simulink model "EvitarObstaculo"  (R2023b)
settings: Solver=FixedStepAuto  StartTime=0.0  StopTime=100.0  FixedStep=Ts  RelTol=1e-3
values from neighbouring files (symbols this model uses):
  obsx = 2    [EjecutarEsquivarObs.m]    (also in EjecutarEsquivarObs_traj.m = 1.75)
  obsy = 0    [EjecutarEsquivarObs.m]    (also in EjecutarEsquivarObs_traj.m = 0.7)
  refx = 10*rand-5    [EjecutarBorroso.m]    (also in EjecutarEsquivarObs.m = 4)
  refy = 10*rand-5    [EjecutarBorroso.m]    (also in EjecutarEsquivarObs.m = 0)
undefined symbols (not defined in the file or in its folder): DiscIntNeverNeededParam
libraries: fuzblock x1
settings Model: Creator=perez  LastModifiedBy=tizia
settings DataIOCC: ReturnWorkspaceOutputs=off

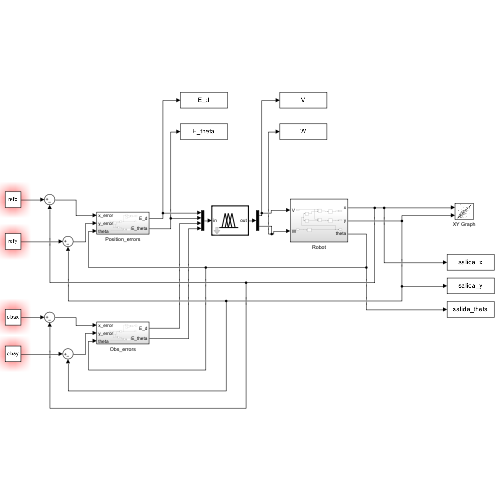
[thumbnail: Simulink's stored preview of the top-level diagram]
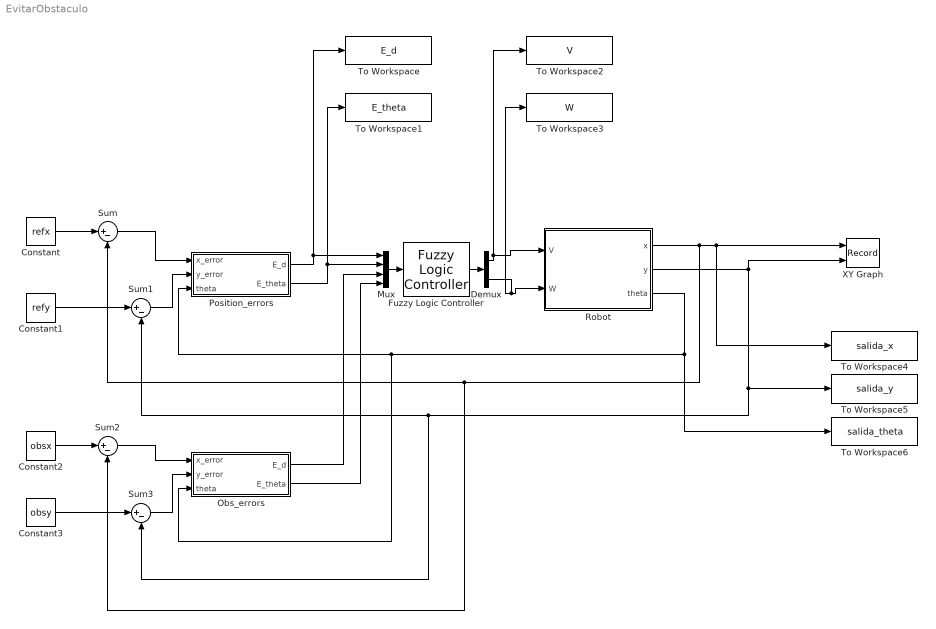
== system EvitarObstaculo ==
  Constant : Constant  Value=refx
  Constant1 : Constant  Value=refy
  Constant2 : Constant  Value=obsx
  Constant3 : Constant  Value=obsy
  Demux : Demux  Outputs=2
  Fuzzy Logic Controller : fuzblock/Fuzzy Logic  Controller  FIS='ControlBorrosoObs.fis'  OutputSampleNumber=101  DataType=double  FuzzifiedInputs=off  RuleFiringStrengths=off  RuleOutputs=off  AggregatedOutputs=off  SimulateUsing=Interpreted execution  OutOfRangeInputValueMessage=warning  NoRuleFiredMessage=warning  EmptyOutputFuzzySetMessage=warning
  Mux : Mux
  Obs_errors : Subsystem
  Position_errors : Subsystem
  Robot : Subsystem
  Sum{,1..3} (4 alike) : Sum  Inputs=|+-
  To Workspace : ToWorkspace  VariableName=E_d  SaveFormat=Structure With Time  SampleTime=-1
  To Workspace1 : ToWorkspace  VariableName=E_theta  SaveFormat=Structure With Time  SampleTime=-1
  To Workspace2 : ToWorkspace  VariableName=V  SaveFormat=Structure With Time  SampleTime=-1
  To Workspace3 : ToWorkspace  VariableName=W  SaveFormat=Structure With Time  SampleTime=-1
  To Workspace4 : ToWorkspace  VariableName=salida_x  SaveFormat=Structure With Time  SampleTime=-1
  To Workspace5 : ToWorkspace  VariableName=salida_y  SaveFormat=Structure With Time  SampleTime=-1
  To Workspace6 : ToWorkspace  VariableName=salida_theta  SaveFormat=Structure With Time  SampleTime=-1
  XY Graph : Record  FileSettingsInternal="{\"entries\":[{\"content\":{\"excelSettings\":{\"content\":{},\"type\":\"Streamout.ExcelSettings\"}},\"type\":\"Streamout.FileSettingStorage\",\"uuid\":\"\"}],\"packageUris\":[\"http:\\/\\/schema.mathworks.com\\/mf0\\/streamout_blocks\\/R2020a\"],\"version\":\"1.0\"}"  Layout=[1 1]  SignalsInternal="{\"entries\":[{\"content\":{\"signals\":[{\"content\":{\"blockPath\":[],\"dimensions\":[1],\"domain\":\"\",\"lineColor\":\"#a2142f\",\"plots\":[ 1 ],\"port\":1,\"signalID\":1,\"signalName\":\"Robot:1\"},\"type\":\"RecordBlkView.Signal\",\"uuid\":\"\"},{\"content\":{\"blockPath\":[],\"dimensions\":[1],\"domain\":\"\",\"lineColor\":\"#139fff\",\"plots\":[ 1 ],\"port\":2,\"signalID\":2,\"signalName\":\"Robot:2\"},\"type\":\"RecordBlkView.Signal\",\"uuid\":\"\"}]},\"type\":\"RecordBlkView.InputSignals\",\"uuid\":\"\"}],\"packageUris\":[\"http:\\/\\/schema.mathworks.com\\/mf0\\/streamout_blocks\\/R2020a\"],\"version\":\"1.0\"}"  VisualizationBindings="{\"xyplotplugin\":{\"info\":[{\"series\":[{\"bindingParametersList\":[{\"parameter\":\"X-Axis\",\"signalID\":1,\"signalName\":\"Robot:1\"},{\"parameter\":\"Y-Axis\",\"signalID\":2,\"signalName\":\"Robot:2\"}],\"seriesID\":0}],\"subplotID\":1}]}}"  CompatibilityTag=XY
  wires:
  Constant/1 -> Sum/1
  Sum/1 -> Position_errors/1(x_error)
  Sum1/1 -> Position_errors/2(y_error)
  Position_errors/1(E_d) -> Mux/1, To Workspace/1
  Position_errors/2(E_theta) -> Mux/2, To Workspace1/1
  Demux/1 -> To Workspace2/1, Robot/1(V)
  Demux/2 -> To Workspace3/1, Robot/2(W)
  Robot/1(x) -> Sum2/2, Sum/2, To Workspace4/1, XY Graph/1
  Robot/2(y) -> To Workspace5/1, Sum3/2, Sum1/2, XY Graph/2
  Robot/3(theta) -> To Workspace6/1, Obs_errors/3(theta), Position_errors/3(theta)
  Constant1/1 -> Sum1/1
  Mux/1 -> Fuzzy Logic Controller/1
  Fuzzy Logic Controller/1 -> Demux/1
  Constant2/1 -> Sum2/1
  Constant3/1 -> Sum3/1
  Sum2/1 -> Obs_errors/1(x_error)
  Sum3/1 -> Obs_errors/2(y_error)
  Obs_errors/1(E_d) -> Mux/3
  Obs_errors/2(E_theta) -> Mux/4

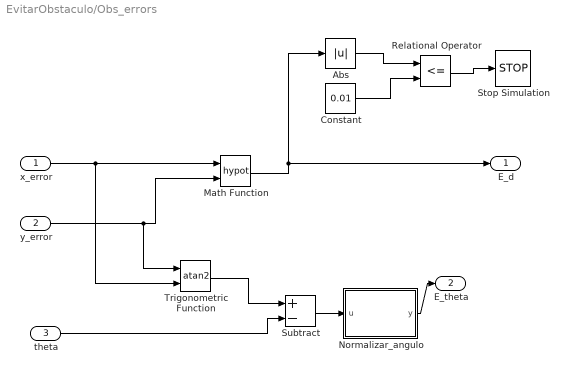
== system EvitarObstaculo/Obs_errors ==
  x_error : Inport
  y_error : Inport  Port=2
  theta : Inport  Port=3
  Abs : Abs  SaturateOnIntegerOverflow=off
  Constant : Constant  Value=0.01
  Math Function : Math  Operator=hypot
  Normalizar_angulo : MATLAB Function  TreatAsAtomicUnit=on
  Relational Operator : RelationalOperator  Operator=<=  OutDataTypeStr=boolean  RndMeth=Simplest  InputSameDT=off
  Stop Simulation : Stop
  Subtract : Sum  Inputs=+-
  Trigonometric Function : Trigonometry  Operator=atan2
  E_d : Outport
  E_theta : Outport  Port=2
  wires:
  x_error/1 -> Trigonometric Function/2, Math Function/1
  y_error/1 -> Trigonometric Function/1, Math Function/2
  Trigonometric Function/1 -> Subtract/1
  theta/1 -> Subtract/2
  Subtract/1 -> Normalizar_angulo/1(u)
  Normalizar_angulo/1(y) -> E_theta/1
  Abs/1 -> Relational Operator/1
  Constant/1 -> Relational Operator/2
  Math Function/1 -> E_d/1, Abs/1
  Relational Operator/1 -> Stop Simulation/1

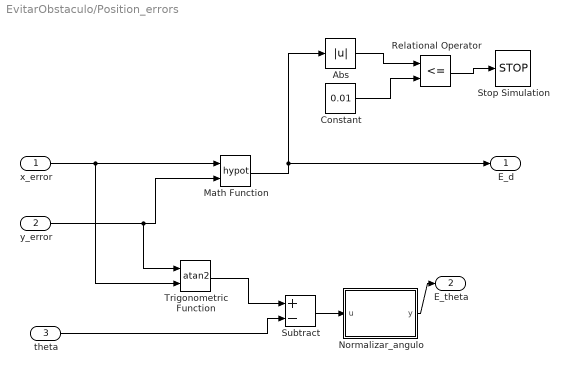
== system EvitarObstaculo/Position_errors ==
  x_error : Inport
  y_error : Inport  Port=2
  theta : Inport  Port=3
  Abs : Abs  SaturateOnIntegerOverflow=off
  Constant : Constant  Value=0.01
  Math Function : Math  Operator=hypot
  Normalizar_angulo : MATLAB Function  TreatAsAtomicUnit=on
  Relational Operator : RelationalOperator  Operator=<=  OutDataTypeStr=boolean  RndMeth=Simplest  InputSameDT=off
  Stop Simulation : Stop
  Subtract : Sum  Inputs=+-
  Trigonometric Function : Trigonometry  Operator=atan2
  E_d : Outport
  E_theta : Outport  Port=2
  wires:
  x_error/1 -> Trigonometric Function/2, Math Function/1
  y_error/1 -> Trigonometric Function/1, Math Function/2
  Trigonometric Function/1 -> Subtract/1
  theta/1 -> Subtract/2
  Subtract/1 -> Normalizar_angulo/1(u)
  Normalizar_angulo/1(y) -> E_theta/1
  Abs/1 -> Relational Operator/1
  Constant/1 -> Relational Operator/2
  Math Function/1 -> E_d/1, Abs/1
  Relational Operator/1 -> Stop Simulation/1

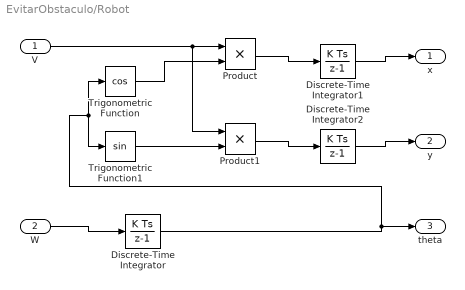
== system EvitarObstaculo/Robot ==
  V : Inport
  W : Inport  Port=2
  Discrete-Time Integrator : DiscreteIntegrator  SampleTime=-1  ICPrevOutput=DiscIntNeverNeededParam  ICPrevScaledInput=DiscIntNeverNeededParam
  Discrete-Time Integrator1 : DiscreteIntegrator  SampleTime=-1  ICPrevOutput=DiscIntNeverNeededParam  ICPrevScaledInput=DiscIntNeverNeededParam
  Discrete-Time Integrator2 : DiscreteIntegrator  SampleTime=-1  ICPrevOutput=DiscIntNeverNeededParam  ICPrevScaledInput=DiscIntNeverNeededParam
  Product : Product
  Product1 : Product
  Trigonometric Function : Trigonometry  Operator=cos
  Trigonometric Function1 : Trigonometry
  x : Outport
  y : Outport  Port=2
  theta : Outport  Port=3
  wires:
  Trigonometric Function1/1 -> Product1/2
  Discrete-Time Integrator2/1 -> y/1
  Discrete-Time Integrator1/1 -> x/1
  Product/1 -> Discrete-Time Integrator1/1
  Product1/1 -> Discrete-Time Integrator2/1
  V/1 -> Product1/1, Product/1
  Discrete-Time Integrator/1 -> Trigonometric Function1/1, Trigonometric Function/1, theta/1
  Trigonometric Function/1 -> Product/2
  W/1 -> Discrete-Time Integrator/1

== matlab function EvitarObstaculo/Position_errors/Normalizar_angulo ==
  data: u input; y output
function y = fcn(u)
% Lleva el ángulo u (rad) a su equivalente en [-pi, pi):
% +pi pasa el intervalo a [0, 2pi), mod quita las vueltas completas
% (también con u negativo) y -pi lo devuelve al intervalo original
y = mod(u + pi, 2*pi) - pi;

== matlab function EvitarObstaculo/Obs_errors/Normalizar_angulo ==
  data: u input; y output
function y = fcn(u)
% Lleva el ángulo u (rad) a su equivalente en [-pi, pi):
% +pi pasa el intervalo a [0, 2pi), mod quita las vueltas completas
% (también con u negativo) y -pi lo devuelve al intervalo original
y = mod(u + pi, 2*pi) - pi;
